simulink model "Sistemas"  (R2026b)
settings: Solver=ode15s  StopTime=10  MaxStep=1E-2
libraries: fl_lib x14, nesl_utility x6, slpidlib x1
settings Model: Creator=demil  LastModifiedBy=19ram
settings SolverCC: AlgebraicLoopSolver=LineSearch
settings DataIOCC: DSMLogging=off  ReturnWorkspaceOutputs=off  SaveOutput=off  SignalLogging=off  TimeSaveName=t
settings DebuggingCC: AlgebraicLoopMsg=none  ArtificialAlgebraicLoopMsg=none  MaxConsecutiveZCsMsg=none  OperatingPointInterfaceChecksumMismatchMsg=none
settings RTWCC: DLArmComputeVersion=19.05
settings SimscapeCC: SimscapeUseEnergyAccounting=off

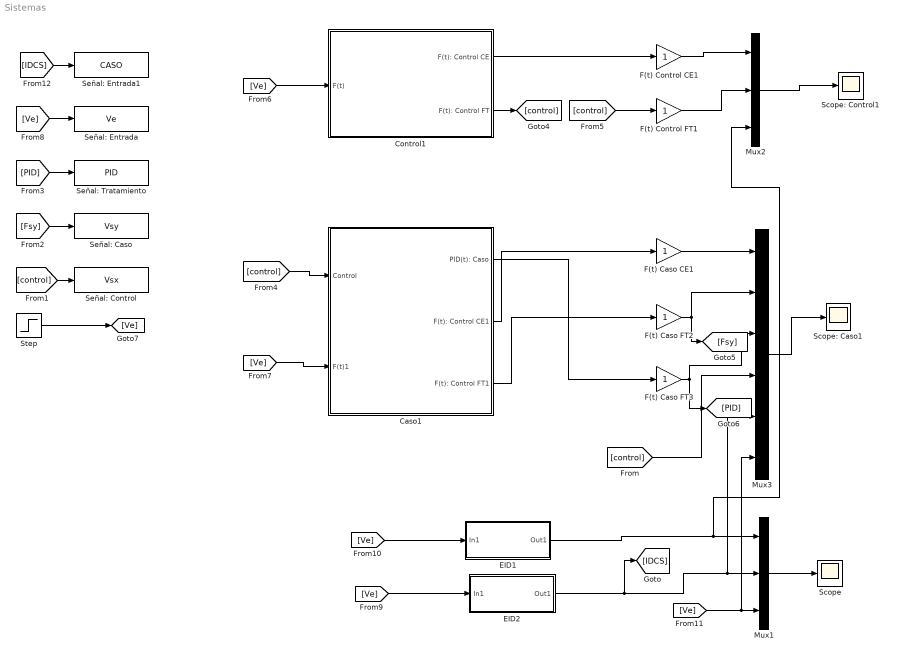
== system Sistemas ==
  Caso1 : Subsystem
  Control1 : Subsystem
  EID1 : Subsystem
  EID2 : Subsystem
  F(t) Caso CE1 : Gain
  F(t) Caso FT2 : Gain
  F(t) Caso FT3 : Gain
  F(t) Control CE1 : Gain
  F(t) Control FT1 : Gain
  Mux1 : Mux  Inputs=3
  Mux2 : Mux  Inputs=3
  Mux3 : Mux  Inputs=6
  Scope : Scope
      settings: ActiveDisplayYMinimum=-0.12376241874880377  ActiveDisplayYMaximum=1.1138617687392343  DataLoggingVariableName=ScopeData2
  Scope: Caso1 : Scope
      settings: ActiveDisplayYMinimum=0.013733941354816204  ActiveDisplayYMaximum=1.1775761566726328
  Scope: Control1 : Scope
      settings: ActiveDisplayYMinimum=-0.066728214532645769  ActiveDisplayYMaximum=1.1066764337257879
  Señal: Caso : ToWorkspace  VariableName=Vsy  SampleTime=-1
  Señal: Control : ToWorkspace  VariableName=Vsx  SampleTime=-1
  Señal: Entrada : ToWorkspace  VariableName=Ve  SampleTime=-1
  Señal: Entrada1 : ToWorkspace  VariableName=CASO  SampleTime=-1
  Señal: Tratamiento : ToWorkspace  VariableName=PID  SampleTime=-1
  Step : Step  Time=0  InitialValue=1  SampleTime=0
  wires:
  [Ve] -> Señal: Entrada/1
  F(t) Control FT1/1 -> Mux2/2
  [PID] -> Señal: Tratamiento/1
  Caso1/1(PID(t): Caso) -> F(t) Caso FT3/1
  [Fsy] -> Señal: Caso/1
  [control] -> Señal: Control/1
  F(t) Caso FT3/1 -> [PID], Mux3/3
  Control1/1(F(t): Control CE) -> F(t) Control CE1/1
  [Ve] -> Control1/1(F(t))
  Control1/2(F(t): Control FT) -> [control]
  F(t) Caso CE1/1 -> Mux3/1
  Step/1 -> [Ve]
  [control] -> Caso1/1(Control)
  Mux3/1 -> Scope: Caso1/1
  F(t) Control CE1/1 -> Mux2/1
  F(t) Caso FT2/1 -> [Fsy], Mux3/2
  [control] -> F(t) Control FT1/1
  Mux2/1 -> Scope: Control1/1
  [Ve] -> Caso1/2(F(t)1)
  Caso1/2(F(t): Control CE1) -> F(t) Caso CE1/1
  Caso1/3(F(t): Control FT1) -> F(t) Caso FT2/1
  [control] -> Mux3/4
  Mux1/1 -> Scope/1
  [Ve] -> EID1/1(In1)
  EID1/1(Out1) -> Mux2/3, Mux1/1
  [Ve] -> EID2/1(In1)
  EID2/1(Out1) -> [IDCS], Mux3/5, Mux1/2
  [Ve] -> Mux3/6, Mux1/3
  [IDCS] -> Señal: Entrada1/1

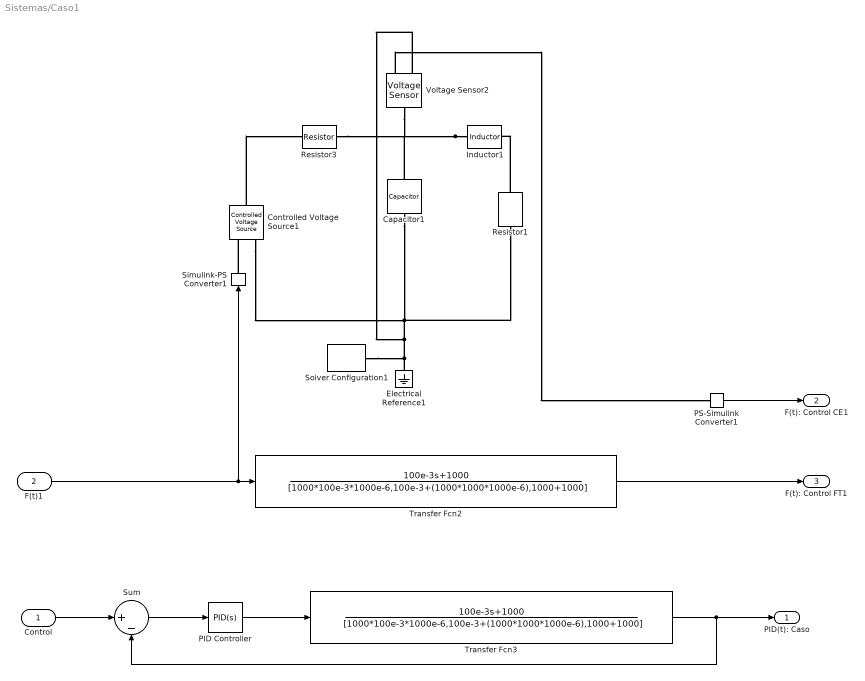
== system Sistemas/Caso1 ==
  Control : Inport
  F(t)1 : Inport  Port=2
  Capacitor1 : fl_lib/Electrical/Electrical Elements/Capacitor  c=1000 uF  r=1e-6 Ohm  g=0 1/Ohm  i_specify=off  i_priority=None  i=0 A  i_nominal_specify=off  i_nominal_value=1  i_nominal_unit=A  v_specify=off  v_priority=None  v=0 V  v_nominal_specify=off  v_nominal_value=1  v_nominal_unit=V  vc_specify=off  vc_priority=High  vc=0 V  vc_nominal_specify=off  vc_nominal_value=1  vc_nominal_unit=V
  Controlled Voltage Source1 : fl_lib/Electrical/Electrical Sources/Controlled Voltage Source
  Electrical Reference1 : fl_lib/Electrical/Electrical Elements/Electrical Reference
  Inductor1 : fl_lib/Electrical/Electrical Elements/Inductor  l=100 mH  r=0 Ohm  g=1e-9 1/Ohm  i_specify=off  i_priority=None  i=0 A  i_nominal_specify=off  i_nominal_value=1  i_nominal_unit=A  v_specify=off  v_priority=None  v=0 V  v_nominal_specify=off  v_nominal_value=1  v_nominal_unit=V  i_L_specify=off  i_L_priority=High  i_L=0 A  i_L_nominal_specify=off  i_L_nominal_value=1  i_L_nominal_unit=A
  PID Controller : slpidlib/PID Controller  Controller=PID  Form=Parallel  TimeDomain=Continuous-time  UseExternalTs=off  SampleTime=-1  IntegratorMethod=Forward Euler  FilterMethod=Forward Euler  ControllerParametersSource=internal  P=1298.69891573232  I=312346.172472053  UseKiTs=off  D=0.179681987650028  UseExternalDerivativeSource=off  N=4964.0941464465  UseFilter=on  TunerSelectOption=Transfer Function Based (PID Tuner App)  InitialConditionSource=internal  InitialConditionForIntegrator=0  InitialConditionForFilter=0  DifferentiatorICPrevScaledInput=0  ExternalReset=none  TrackingMode=off  Kt=1  LimitOutput=off  SatLimitsSource=internal  UpperSaturationLimit=inf  LowerSaturationLimit=-inf  LinearizeAsGain=on  AntiWindupMode=none  Kb=1  LimitIntegrator=off  UpperIntegratorSaturationLimit=inf  LowerIntegratorSaturationLimit=-inf  POutMin=[]  POutMax=[]  IOutMin=[]  IOutMax=[]  DOutMin=[]  DOutMax=[]  NOutMin=[]  NOutMax=[]  SumOutMin=[]  SumOutMax=[]  SaturationOutMin=[]  SaturationOutMax=[]  PParamMin=[]  PParamMax=[]  IParamMin=[]  IParamMax=[]  DParamMin=[]  DParamMax=[]  NParamMin=[]  NParamMax=[]  KbParamMin=[]  KbParamMax=[]  KtParamMin=[]  KtParamMax=[]  KbOutMin=[]  KbOutMax=[]  KtOutMin=[]  KtOutMax=[]  IntegratorOutMin=[]  IntegratorOutMax=[]  FilterOutMin=[]  FilterOutMax=[]  SumI1OutMin=[]  SumI1OutMax=[]  SumI2OutMin=[]  SumI2OutMax=[]  SumI3OutMin=[]  SumI3OutMax=[]  SumI4OutMin=[]  SumI4OutMax=[]  SumDOutMin=[]  SumDOutMax=[]  DifferentiatorOutMin=[]  DifferentiatorOutMax=[]  FilterDiffOutCoefMin=[]  FilterDiffOutCoefMax=[]  ReciprocalOutMin=[]  ReciprocalOutMax=[]  SumDenOutMin=[]  SumDenOutMax=[]  SumNumOutMin=[]  SumNumOutMax=[]  DivideOutMin=[]  DivideOutMax=[]  UdiffTsProdOutMin=[]  UdiffTsProdOutMax=[]  NTsProdOutMin=[]  NTsProdOutMax=[]  UintegralTsProdOutMin=[]  UintegralTsProdOutMax=[]  UngainTsProdOutMin=[]  UngainTsProdOutMax=[]  ClampingZeroOutDataTypeStr=Inherit: Inherit via back propagation  ClampingZeroOutMin=[]  ClampingZeroOutMax=[]  FilterDenConstantOutDataTypeStr=Inherit: Inherit via back propagation  FilterDenConstantOutMin=[]  FilterDenConstantOutMax=[]  PCopyOutDataTypeStr=Inherit: Inherit via back propagation  PCopyOutMin=[]  PCopyOutMax=[]  NCopyOutDataTypeStr=Inherit: Inherit via back propagation  NCopyOutMin=[]  NCopyOutMax=[]  IntegratorContinuousStateAttributes=''  IntegratorStateMustResolveToSignalObject=off  IntegratorRTWStateStorageClass=Auto  FilterContinuousStateAttributes=''  FilterStateMustResolveToSignalObject=off  FilterRTWStateStorageClass=Auto  ParallelPVariant=InternalParameters  IdealPVariant=Disabled  IVariant=InternalParameters  DVariant=InternalParameters  IntegratorVariant=Continuous  SatVariant=Disabled  AWVariant=Passthrough  PCopyVariant=Disabled  TRVariant=Disabled  FdbkBlocksVariant=Forward  IdealPFdbkVariant=Disabled  SatFdbkVariant=Disabled  DerivativeFilterVariant=ContFilter  NVariant=InternalParameters  NCopyVariant=Disabled  FilterICVariant=InternalICsFilter  IntegratorICVariant=InternalICs  ExternalResetVariant=Disabled  TRSumVariant=Passthrough  SumFdbkVariant=Disabled  SumVariant=Sum_PID  TsampFilterVariant=InternalTs  TsampNgainVariant=Passthrough  TsampIntegralVariant=Disabled_SignalSpec  ExternalSaturationOutDataTypeStr=Inherit: Same as second input  DerivativeSourceVariant=ErrorSignal  PreIntVariant=InternalPreInt
  PS-Simulink Converter1 : nesl_utility/PS-Simulink Converter  PhysicalDomain=network_engine_domain  SubClassName=ps_output  LeftPortType=input  RightPortType=output  PseudoPeriodic=off  Frequencies=[]  VectorFormat=1-D array  Unit=inherit  AffineConversion=off
  Resistor1 : fl_lib/Electrical/Electrical Elements/Resistor  R=1 kOhm  i_specify=off  i_priority=None  i=0 A  i_nominal_specify=off  i_nominal_value=1  i_nominal_unit=A  v_specify=off  v_priority=None  v=0 V  v_nominal_specify=off  v_nominal_value=1  v_nominal_unit=V
  Resistor3 : fl_lib/Electrical/Electrical Elements/Resistor  R=1 kOhm  i_specify=off  i_priority=None  i=0 A  i_nominal_specify=off  i_nominal_value=1  i_nominal_unit=A  v_specify=off  v_priority=None  v=0 V  v_nominal_specify=off  v_nominal_value=1  v_nominal_unit=V
  Simulink-PS Converter1 : nesl_utility/Simulink-PS Converter  PhysicalDomain=network_engine_domain  SubClassName=ps_input  LeftPortType=input  RightPortType=output  PseudoPeriodic=off  Frequencies=[]  NoiseDistribution=none  NoiseParameters=[]  Unit=1  AffineConversion=off  FilteringAndDerivatives=provide  SimscapeFilterOrder=1  InputFilterTimeConstant=0.001  UdotUserProvided=0
  Solver Configuration1 : nesl_utility/Solver Configuration  PhysicalDomain=network_engine_domain  SubClassName=solver  LeftPortType=input  RightPortType=generic  Tones=[]  Harmonics=[]  SimulateNoise=off  Profile=off  UseLocalSampling=off  EnableSwitchedLinearOptims=on  FrequencyDomain=off  UseCCode=off  RelTol=0.001  AbsTol=0.001  MinStep=1e-09  ToWorkspace=off  RevertToSquareIcSolve=off  NumHomotopyIterations=100  PhasorMode=off  PhasorModeNumHarmonics=1  ConsistencySolver=NEWTON_XTOL_AFTER_FTOL  CanonicalOrdering=CANONICAL  OptimizeIntermediates=OPTIMIZED  MulticoreSolverChoice=BACKWARD_EULER  IndexReductionMethod=DerivativeReplacement  DoDC=off  ResidualTolerance=1e-09  ConsistencyTolSource=GLOBAL  ConsistencyAbsTol=0.001  ConsistencyRelTol=0.001  ConsistencyTolFactor=0.001  UseLocalSolver=off  LocalSolverChoice=NE_BACKWARD_EULER_ADVANCER  ResolveIndetEquations=on  FunctionEvalNumThread=1  LocalSolverSampleTime=0.001  DoFixedCost=off  MaxNonlinIter=3  MaxModeIter=2  ComputeImpulses=off  ImpulseIterations=2  LinearAlgebra=auto  LinearAlgebraNumThread=0  EquationFormulation=NE_TIME_EF  DelaysMemoryBudget=1024  AutomaticFiltering=on  FilteringTimeConstant=0.001  PartitionStorageMethod=AS_NEEDED  PartitionMemoryBudget=1024  PartitionMethod=BALANCED  MultibodyUseLocalSolver=off  MultibodyLocalSolverChoice=ODE1  MultibodyLocalSolverSampleTime=0.001
  Sum : Sum  Inputs=|+-
  Transfer Fcn2 : TransferFcn  Numerator=[100e-3,1000]  Denominator=[1000*100e-3*1000e-6,100e-3+(1000*1000*1000e-6),1000+1000]
  Transfer Fcn3 : TransferFcn  Numerator=[100e-3,1000]  Denominator=[1000*100e-3*1000e-6,100e-3+(1000*1000*1000e-6),1000+1000]
  Voltage Sensor2 : fl_lib/Electrical/Electrical Sensors/Voltage Sensor
  PID(t): Caso : Outport
  F(t): Control CE1 : Outport  Port=2
  F(t): Control FT1 : Outport  Port=3
  wires:
  Control/1 -> Sum/1
  Sum/1 -> PID Controller/1
  PID Controller/1 -> Transfer Fcn3/1
  Transfer Fcn3/1 -> PID(t): Caso/1, Sum/2
  F(t)1/1 -> Simulink-PS Converter1/1, Transfer Fcn2/1
  PS-Simulink Converter1/1 -> F(t): Control CE1/1
  Transfer Fcn2/1 -> F(t): Control FT1/1
  connections:
  Electrical Reference1/LConn1 -- Solver Configuration1/RConn1 -- Voltage Sensor2/RConn2 -- Resistor1/RConn1 -- Capacitor1/RConn1 -- Controlled Voltage Source1/RConn2
  Inductor1/LConn1 -- Voltage Sensor2/LConn1 -- Capacitor1/LConn1 -- Resistor3/RConn1
  Controlled Voltage Source1/LConn1 -- Resistor3/LConn1
  Simulink-PS Converter1/RConn1 -- Controlled Voltage Source1/RConn1
  Voltage Sensor2/RConn1 -- PS-Simulink Converter1/LConn1
  Resistor1/LConn1 -- Inductor1/RConn1

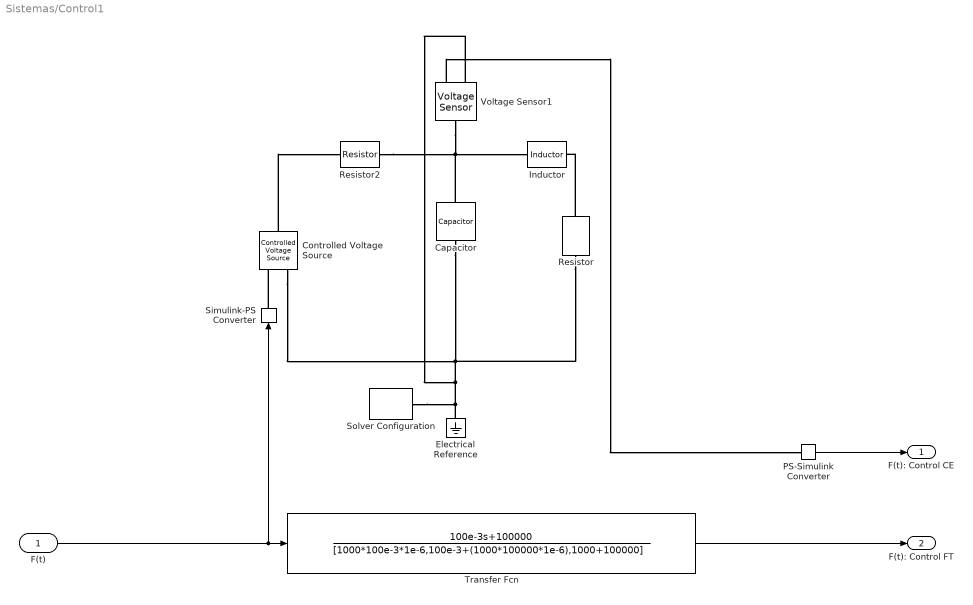
== system Sistemas/Control1 ==
  F(t) : Inport
  Capacitor : fl_lib/Electrical/Electrical Elements/Capacitor  c=1 uF  r=1e-6 Ohm  g=0 1/Ohm  i_specify=off  i_priority=None  i=0 A  i_nominal_specify=off  i_nominal_value=1  i_nominal_unit=A  v_specify=off  v_priority=None  v=0 V  v_nominal_specify=off  v_nominal_value=1  v_nominal_unit=V  vc_specify=off  vc_priority=High  vc=0 V  vc_nominal_specify=off  vc_nominal_value=1  vc_nominal_unit=V
  Controlled Voltage Source : fl_lib/Electrical/Electrical Sources/Controlled Voltage Source
  Electrical Reference : fl_lib/Electrical/Electrical Elements/Electrical Reference
  Inductor : fl_lib/Electrical/Electrical Elements/Inductor  l=100 mH  r=0 Ohm  g=1e-9 1/Ohm  i_specify=off  i_priority=None  i=0 A  i_nominal_specify=off  i_nominal_value=1  i_nominal_unit=A  v_specify=off  v_priority=None  v=0 V  v_nominal_specify=off  v_nominal_value=1  v_nominal_unit=V  i_L_specify=off  i_L_priority=High  i_L=0 A  i_L_nominal_specify=off  i_L_nominal_value=1  i_L_nominal_unit=A
  PS-Simulink Converter : nesl_utility/PS-Simulink Converter  PhysicalDomain=network_engine_domain  SubClassName=ps_output  LeftPortType=input  RightPortType=output  PseudoPeriodic=off  Frequencies=[]  VectorFormat=1-D array  Unit=inherit  AffineConversion=off
  Resistor : fl_lib/Electrical/Electrical Elements/Resistor  R=100 kOhm  i_specify=off  i_priority=None  i=0 A  i_nominal_specify=off  i_nominal_value=1  i_nominal_unit=A  v_specify=off  v_priority=None  v=0 V  v_nominal_specify=off  v_nominal_value=1  v_nominal_unit=V
  Resistor2 : fl_lib/Electrical/Electrical Elements/Resistor  R=1000 Ohm  i_specify=off  i_priority=None  i=0 A  i_nominal_specify=off  i_nominal_value=1  i_nominal_unit=A  v_specify=off  v_priority=None  v=0 V  v_nominal_specify=off  v_nominal_value=1  v_nominal_unit=V
  Simulink-PS Converter : nesl_utility/Simulink-PS Converter  PhysicalDomain=network_engine_domain  SubClassName=ps_input  LeftPortType=input  RightPortType=output  PseudoPeriodic=off  Frequencies=[]  NoiseDistribution=none  NoiseParameters=[]  Unit=1  AffineConversion=off  FilteringAndDerivatives=provide  SimscapeFilterOrder=1  InputFilterTimeConstant=0.001  UdotUserProvided=0
  Solver Configuration : nesl_utility/Solver Configuration  PhysicalDomain=network_engine_domain  SubClassName=solver  LeftPortType=input  RightPortType=generic  Tones=[]  Harmonics=[]  SimulateNoise=off  Profile=off  UseLocalSampling=off  EnableSwitchedLinearOptims=on  FrequencyDomain=off  UseCCode=off  RelTol=0.001  AbsTol=0.001  MinStep=1e-09  ToWorkspace=off  RevertToSquareIcSolve=off  NumHomotopyIterations=100  PhasorMode=off  PhasorModeNumHarmonics=1  ConsistencySolver=NEWTON_XTOL_AFTER_FTOL  CanonicalOrdering=CANONICAL  OptimizeIntermediates=OPTIMIZED  MulticoreSolverChoice=BACKWARD_EULER  IndexReductionMethod=DerivativeReplacement  DoDC=off  ResidualTolerance=1e-09  ConsistencyTolSource=GLOBAL  ConsistencyAbsTol=0.001  ConsistencyRelTol=0.001  ConsistencyTolFactor=0.001  UseLocalSolver=off  LocalSolverChoice=NE_BACKWARD_EULER_ADVANCER  ResolveIndetEquations=on  FunctionEvalNumThread=1  LocalSolverSampleTime=0.001  DoFixedCost=off  MaxNonlinIter=3  MaxModeIter=2  ComputeImpulses=off  ImpulseIterations=2  LinearAlgebra=auto  LinearAlgebraNumThread=0  EquationFormulation=NE_TIME_EF  DelaysMemoryBudget=1024  AutomaticFiltering=on  FilteringTimeConstant=0.001  PartitionStorageMethod=AS_NEEDED  PartitionMemoryBudget=1024  PartitionMethod=BALANCED  MultibodyUseLocalSolver=off  MultibodyLocalSolverChoice=ODE1  MultibodyLocalSolverSampleTime=0.001
  Transfer Fcn : TransferFcn  Numerator=[100e-3,100000]  Denominator=[1000*100e-3*1e-6,100e-3+(1000*100000*1e-6),1000+100000]
  Voltage Sensor1 : fl_lib/Electrical/Electrical Sensors/Voltage Sensor
  F(t): Control CE : Outport
  F(t): Control FT : Outport  Port=2
  wires:
  F(t)/1 -> Simulink-PS Converter/1, Transfer Fcn/1
  PS-Simulink Converter/1 -> F(t): Control CE/1
  Transfer Fcn/1 -> F(t): Control FT/1
  connections:
  Simulink-PS Converter/RConn1 -- Controlled Voltage Source/RConn1
  Electrical Reference/LConn1 -- Solver Configuration/RConn1 -- Voltage Sensor1/RConn2 -- Resistor/RConn1 -- Capacitor/RConn1 -- Controlled Voltage Source/RConn2
  Voltage Sensor1/RConn1 -- PS-Simulink Converter/LConn1
  Controlled Voltage Source/LConn1 -- Resistor2/LConn1
  Resistor2/RConn1 -- Voltage Sensor1/LConn1 -- Capacitor/LConn1 -- Inductor/LConn1
  Resistor/LConn1 -- Inductor/RConn1

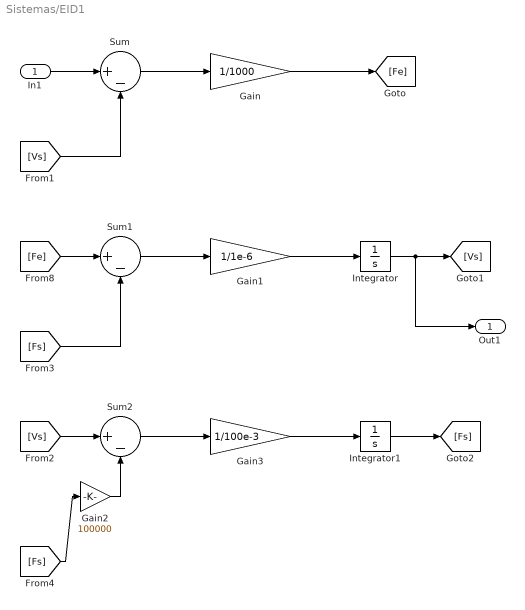
== system Sistemas/EID1 ==
  In1 : Inport
  Gain : Gain  Gain=1/1000
  Gain1 : Gain  Gain=1/1e-6
  Gain2 : Gain  Gain=100000
  Gain3 : Gain  Gain=1/100e-3
  Integrator : Integrator
  Integrator1 : Integrator
  Sum : Sum  Inputs=|+-
  Sum1 : Sum  Inputs=|+-
  Sum2 : Sum  Inputs=|+-
  Out1 : Outport
  wires:
  In1/1 -> Sum/1
  [Vs] -> Sum/2
  Sum/1 -> Gain/1
  Gain/1 -> [Fe]
  [Fe] -> Sum1/1
  [Fs] -> Sum1/2
  Sum1/1 -> Gain1/1
  Gain1/1 -> Integrator/1
  Integrator/1 -> Out1/1, [Vs]
  [Vs] -> Sum2/1
  [Fs] -> Gain2/1
  Gain2/1 -> Sum2/2
  Sum2/1 -> Gain3/1
  Gain3/1 -> Integrator1/1
  Integrator1/1 -> [Fs]

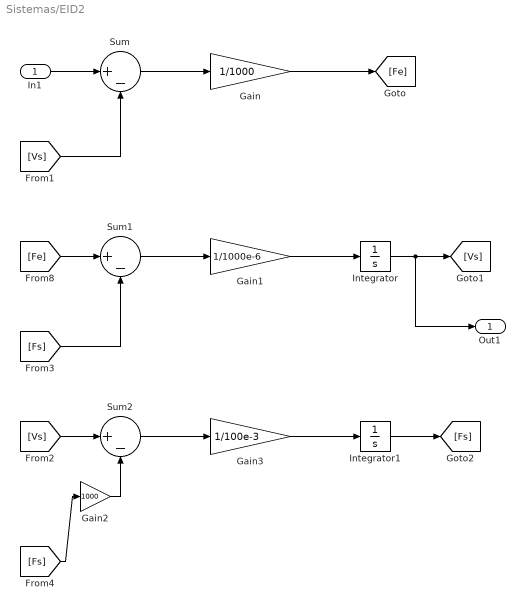
== system Sistemas/EID2 ==
  In1 : Inport
  Gain : Gain  Gain=1/1000
  Gain1 : Gain  Gain=1/1000e-6
  Gain2 : Gain  Gain=1000
  Gain3 : Gain  Gain=1/100e-3
  Integrator : Integrator
  Integrator1 : Integrator
  Sum : Sum  Inputs=|+-
  Sum1 : Sum  Inputs=|+-
  Sum2 : Sum  Inputs=|+-
  Out1 : Outport
  wires:
  In1/1 -> Sum/1
  [Vs] -> Sum/2
  Sum/1 -> Gain/1
  Gain/1 -> [Fe]
  [Fe] -> Sum1/1
  [Fs] -> Sum1/2
  Sum1/1 -> Gain1/1
  Gain1/1 -> Integrator/1
  Integrator/1 -> Out1/1, [Vs]
  [Vs] -> Sum2/1
  [Fs] -> Gain2/1
  Gain2/1 -> Sum2/2
  Sum2/1 -> Gain3/1
  Gain3/1 -> Integrator1/1
  Integrator1/1 -> [Fs]
